simulink model "PrmM"  (R2025b)
settings: Solver=FixedStepDiscrete  StartTime=0.0  StopTime=5  RelTol=1e-3  EnableMultiTasking=on
PreLoadFcn:
  | loaded_model = bdroot;
  | cd (fileparts(get_param(bdroot,'FileName')));
  | SEGInitDevEnv
libraries: ParameterManager x2
settings Model: DataDictionary=PrmM_Data.sldd  EnableAccessToBaseWorkspace=off  Creator=BET2ST  LastModifiedBy=JVE2ST
settings DataIOCC: SaveFormat=StructureWithTime  SaveState=on
settings OptimizationCC: BlockReduction=off  DefaultParameterBehavior=Inlined  UseDivisionForNetSlopeComputation=on  DefaultUnderspecifiedDataType=single  InlineInvariantSignals=on  EnhancedBackFolding=on  PassReuseOutputArgsAs=Individual arguments  RollThreshold=40.0  ActiveStateOutputEnumStorageType=uint8  ZeroExternalMemoryAtStartup=off  EfficientFloat2IntCast=on  LifeSpan=inf  BufferReusableBoundary=off  OptimizeBlockOrder=speed  DifferentSizesBufferReuse=on  OptimizationCustomize=off  LabelGuidedReuse=on  EfficientTunableParamExpr=on
settings DebuggingCC: SignalInfNanChecking=error  SignalRangeChecking=error  ReadBeforeWriteMsg=EnableAllAsError  WriteAfterWriteMsg=EnableAllAsError  WriteAfterReadMsg=EnableAllAsError  AlgebraicLoopMsg=error  ArtificialAlgebraicLoopMsg=error  SaveWithDisabledLinksMsg=error  SaveWithParameterizedLinksMsg=error  BlockPriorityViolationMsg=error  SolverPrmCheckMsg=error  InheritedTsInSrcMsg=error  SingleTaskRateTransMsg=error  TasksWithSamePriorityMsg=error  SigSpecEnsureSampleTimeMsg=error  CheckMatrixSingularityMsg=error  IntegerOverflowMsg=error  ParameterUnderflowMsg=error  ParameterPrecisionLossMsg=error  ParameterTunabilityLossMsg=error  UnderSpecifiedDataTypeMsg=error  UnnecessaryDatatypeConvMsg=warning  VectorMatrixConversionMsg=error  SignalLabelMismatchMsg=error  UnconnectedInputMsg=error  UnconnectedOutputMsg=error  UnconnectedLineMsg=error  SFcnCompatibilityMsg=error  FrameProcessingCompatibilityMsg=warning  UniqueDataStoreMsg=error  BusObjectLabelMismatch=error  RootOutportRequireBusObject=error  AssertControl=DisableAll  AllowSymbolicDim=off  ModelReferenceIOMismatchMessage=error  UnknownTsInhSupMsg=error  ModelReferenceDataLoggingMessage=error  StateNameClashWarn=warning  StrictBusMsg=ErrorOnBusTreatedAsVector  NonBusSignalsTreatedAsBus=error  SFInvalidInputDataAccessInChartInitDiag=error  SFTransitionOutsideNaturalParentDiag=error  SFUnreachableExecutionPathDiag=error  SFUndirectedBroadcastEventsDiag=error  SFTransitionActionBeforeConditionDiag=error  SFTemporalDelaySmallerThanSampleTimeDiag=error  SFSelfTransitionDiag=error  SFExecutionAtInitializationDiag=error  IntegerSaturationMsg=error
settings HardwareCC: ProdBitPerPointer=32.0  ProdBitPerSizeT=32.0  ProdBitPerPtrDiffT=32.0  ProdLargestAtomicInteger=Long  ProdWordSize=32.0  ProdHWDeviceType=Infineon->TriCore
settings ModelReferenceCC: EnableRefExpFcnMdlSchedulingChecks=on  EnableParallelModelReferenceBuilds=on  ModelReferenceNumInstancesAllowed=Single  PropagateSignalLabelsOutOfModel=off
settings SFSimCC: SFSimEcho=off  SimGenImportedTypeDefs=on  CompileTimeRecursionLimit=0.0  EnableRuntimeRecursion=off  MATLABDynamicMemAlloc=off
settings RTWCC: SystemTargetFile=autosar.tlc  GenCodeOnly=on  TemplateMakefile=ert_default_tmf  PostCodeGenCommand=SEGPostCodeGenCallback(modelName, buildInfo)  DataTypeReplacement=CDataTypesFixedWidth  Description=AUTOSAR
settings CodeAppCC: ForceParamTrailComments=on  CommentStyle=Single-line  IgnoreCustomStorageClasses=off  IgnoreTestpoints=on  OperatorAnnotations=on  SimulinkDataObjDesc=on  SFDataObjDesc=on  MATLABFcnDesc=on  MangleLength=4.0  SharedChecksumLength=4.0  CustomSymbolStrGlobalVar=$U$R$N$M  CustomSymbolStrType=$R_$N$M  CustomSymbolStrFcn=$U$R_$N$F$M  CustomSymbolStrFcnArg=$U$N$M_$I[l]  CustomSymbolStrBlkIO=$N$M  InsertBlockDesc=on  StateflowObjectComments=on  MATLABSourceComments=on  ReqsInCode=on
settings STFCustomTargetCC: SystemTargetFile=autosar.tlc  TargetLangStandard=C99 (ISO)  UtilityFuncGeneration=Shared location  MultiwordLength=256.0  ParMdlRefBuildCompliant=on  CompOptLevelCompliant=on  ConcurrentExecutionCompliant=off  IncludeMdlTerminateFcn=off  CombineOutputUpdateFcns=on  SuppressErrorStatus=on  ERTCustomFileBanners=on  SubcomponentCodeInterfacePackaging=Nonreusable function  SupportNonFinite=off  SupportComplex=off  SupportContinuousTime=off  SupportNonInlinedSFcns=off  RemoveResetFunc=on  ParenthesesLevel=Standards  CastingMode=Standards  MATLABClassNameForMDSCustomization=Simulink.SoftwareTarget.ERTCustomization  AutosarCompliant=on  GRTInterface=off  UseToolchainInfoCompliant=on  GenerateSharedConstants=off  LookupTableObjectStructAxisOrder=2,1,3,4,...  LUTObjectStructOrderEvenSpacing=Size,Table,Breakpoints  AutosarSchemaVersion=R23-11  AutosarMaxShortNameLength=128.0  AutosarCompilerAbstraction=off  AutosarMatrixIOAsArray=off  DisableAUTOSARRoutinesHostLibrary=off
settings ERTTargetCC: ERTCustomFileTemplate=example_file_process.tlc  ERTFilePackagingFormat=Compact  PreserveExpressionOrder=on  SuppressUnreachableDefaultCases=off  EnableSignedLeftShifts=off  EnableSignedRightShifts=off  BooleanTrueId=TRUE  BooleanFalseId=FALSE  MemSecPackage=arMemmap  MemSecDataInternal=VAR_UNSPECIFIED  MemSecFuncExecute=CODE  MemSecFuncSharedUtil=CODE  TargetLangStandard=C99 (ISO)  UtilityFuncGeneration=Shared location  ConcurrentExecutionCompliant=off  IncludeMdlTerminateFcn=off  SuppressErrorStatus=on  SubcomponentCodeInterfacePackaging=Nonreusable function  SupportNonFinite=off  SupportComplex=off  ParenthesesLevel=Standards  CastingMode=Standards  ModelStepFunctionPrototypeControlCompliant=off  CPPClassGenCompliant=off  AutosarCompliant=on  GenerateSharedConstants=off  LookupTableObjectStructAxisOrder=2,1,3,4,...  LUTObjectStructOrderEvenSpacing=Size,Table,Breakpoints

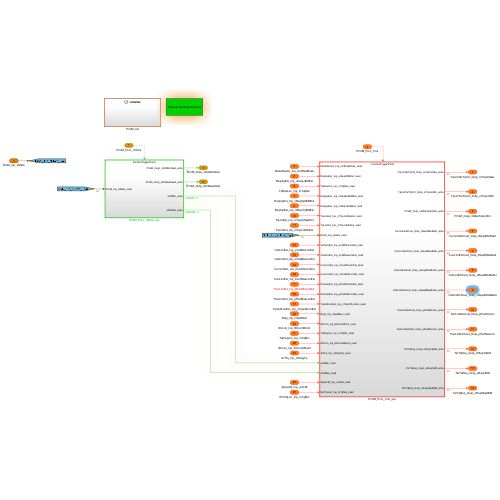
[thumbnail: Simulink's stored preview of the top-level diagram]
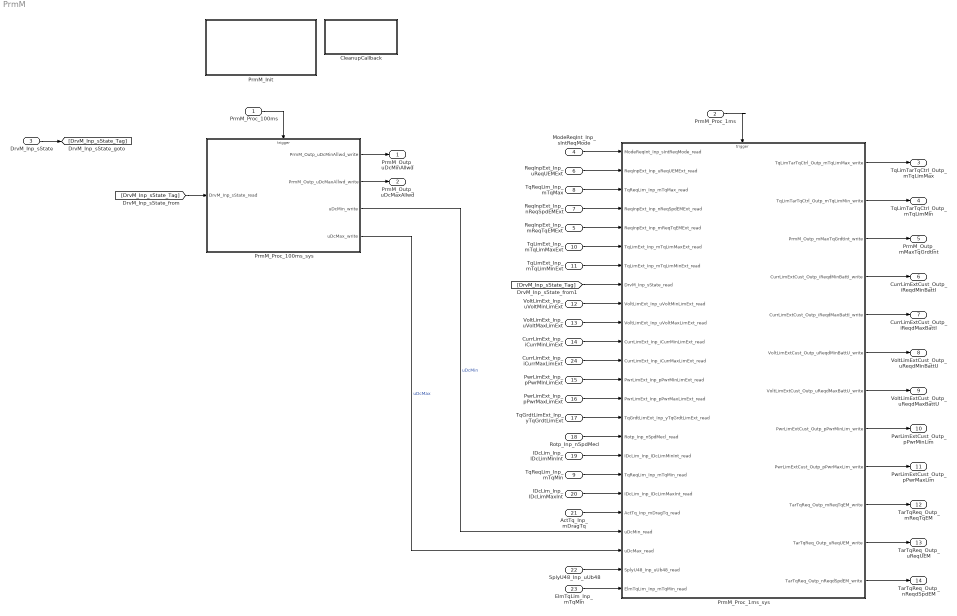
== system PrmM ==
  PrmM_Proc_100ms : Inport  SampleTime=0.1  OutputFunctionCall=on
  PrmM_Proc_1ms : Inport  Port=2  SampleTime=0.001  OutputFunctionCall=on
  DrvM_Inp_sState : Inport  Port=3  OutDataTypeStr=Enum: AD_DrvM_tSTATEIDX_E  PortDimensions=1
  ModeReqInt_Inp_sIntReqMode : Inport  Port=4  OutDataTypeStr=Enum: AD_DrvM_tSTATEIDX_E  PortDimensions=1
  ReqInpExt_Inp_mReqTqEMExt : Inport  Port=5  OutMin=-75  OutMax=75  OutDataTypeStr=AD_tMREQTQEMEXT  PortDimensions=1
  ReqInpExt_Inp_uReqUEMExt : Inport  Port=6  OutMin=0  OutMax=60  OutDataTypeStr=AD_tUREQVOLTEMEXT  PortDimensions=1
  ReqInpExt_Inp_nReqSpdEMExt : Inport  Port=7  OutMin=-10000  OutMax=55534  OutDataTypeStr=AD_tNREQDSPDEMEXT  PortDimensions=1
  TqReqLim_Inp_mTqMax : Inport  Port=8  OutMin=-85  OutMax=85  OutDataTypeStr=AD_TqReqLim_tMTQMAX  PortDimensions=1
  TqReqLim_Inp_mTqMin : Inport  Port=9  OutMin=-85  OutMax=85  OutDataTypeStr=AD_TqReqLim_tMTQMIN  PortDimensions=1
  TqLimExt_Inp_mTqLimMaxExt : Inport  Port=10  OutMin=0  OutMax=65  OutDataTypeStr=AD_tMTQLIMMAXEXT  PortDimensions=1
  TqLimExt_Inp_mTqLimMinExt : Inport  Port=11  OutMin=-65  OutMax=0  OutDataTypeStr=AD_tMTQLIMMINEXT  PortDimensions=1
  VoltLimExt_Inp_uVoltMinLimExt : Inport  Port=12  OutMin=20  OutMax=65  OutDataTypeStr=AD_tUVOLTMINLIMEXT  PortDimensions=1
  VoltLimExt_Inp_uVoltMaxLimExt : Inport  Port=13  OutMin=20  OutMax=65  OutDataTypeStr=AD_tUVOLTMAXLIMEXT  PortDimensions=1
  CurrLimExt_Inp_iCurrMinLimExt : Inport  Port=14  OutMin=-1200  OutMax=1200  OutDataTypeStr=AD_tICURRMINLIMEXT  PortDimensions=1
  PwrLimExt_Inp_pPwrMInLimExt : Inport  Port=15  OutMin=-16000  OutMax=16000  OutDataTypeStr=AD_tPPWRMINLIMEXT  PortDimensions=1
  PwrLimExt_Inp_pPwrMaxLimExt : Inport  Port=16  OutMin=-16000  OutMax=16000  OutDataTypeStr=AD_tPPWRMAXLIMEXT  PortDimensions=1
  TqGrdtLimExt_Inp_yTqGrdtLimExt : Inport  Port=17  OutMin=0  OutMax=2000  OutDataTypeStr=AD_tYTQGRDTLIMEXT  PortDimensions=1
  Rotp_Inp_nSpdMecl : Inport  Port=18  OutMin=-22000  OutMax=22000  OutDataTypeStr=AD_RotP_tNSPDMECL  PortDimensions=1
  IDcLim_Inp_IDcLimMinInt : Inport  Port=19  OutMin=-400  OutMax=0  OutDataTypeStr=AD_tIDCLIMMININT  PortDimensions=1
  IDcLim_Inp_IDcLimMaxInt : Inport  Port=20  OutMin=0  OutMax=400  OutDataTypeStr=AD_tIDCLIMMAXINT  PortDimensions=1
  ActTq_Inp_mDragTq : Inport  Port=21  OutMin=-85  OutMax=85  OutDataTypeStr=AD_ActTq_tMDRAGTQ  PortDimensions=1
  SplyU48_Inp_uUb48 : Inport  Port=22  OutMin=0  OutMax=80  OutDataTypeStr=AD_SplyU_tUUB48  PortDimensions=1
  ElmTqLim_Inp_mTqMin : Inport  Port=23  OutMin=-85  OutMax=0  OutDataTypeStr=AD_ElmTqLim_tMTQMIN  PortDimensions=1
  CurrLimExt_Inp_iCurrMaxLimExt : Inport  Port=24  OutMin=-1200  OutMax=1200  OutDataTypeStr=AD_tICURRMAXLIMEXT  PortDimensions=1
  CleanupCallback : Subsystem
      settings: OpenFcn=SEGCleanWorkspace
      mask Display: disp('Cleanup Working Directory')
  PrmM_Init : Subsystem
  PrmM_Proc_100ms_sys : Subsystem
  PrmM_Proc_1ms_sys : Subsystem
  PrmM_Outp_uDcMinAllwd : Outport  OutMin=20  OutMax=65  OutDataTypeStr=AD_PrmM_tUDCMINALLWD  PortDimensions=1  VectorParamsAs1DForOutWhenUnconnected=off
  PrmM_Outp_uDcMaxAllwd : Outport  Port=2  OutMin=20  OutMax=65  OutDataTypeStr=AD_PrmM_tUDCMAXALLWD  PortDimensions=1  VectorParamsAs1DForOutWhenUnconnected=off
  TqLimTarTqCtrl_Outp_mTqLimMax : Outport  Port=3  OutMin=-75  OutMax=75  OutDataTypeStr=AD_ComWrp_tMTQLIMMAX  PortDimensions=1  VectorParamsAs1DForOutWhenUnconnected=off
  TqLimTarTqCtrl_Outp_mTqLimMin : Outport  Port=4  OutMin=-75  OutMax=75  OutDataTypeStr=AD_ComWrp_tMTQLIMMIN  PortDimensions=1  VectorParamsAs1DForOutWhenUnconnected=off
  PrmM_Outp_mMaxTqGrdtInt : Outport  Port=5  OutMin=0.10000000149011612  OutMax=2000  OutDataTypeStr=AD_PrmM_tMMAXTQGRDINT  PortDimensions=1  VectorParamsAs1DForOutWhenUnconnected=off
  CurrLimExtCust_Outp_iReqdMinBattI : Outport  Port=6  OutMin=-1200  OutMax=1200  OutDataTypeStr=AD_ComWrp_tIREQDMINBATTI  PortDimensions=1  VectorParamsAs1DForOutWhenUnconnected=off
  CurrLimExtCust_Outp_iReqdMaxBattI : Outport  Port=7  OutMin=-1200  OutMax=1200  OutDataTypeStr=AD_ComWrp_tIREQDMAXBATTI  PortDimensions=1  VectorParamsAs1DForOutWhenUnconnected=off
  VoltLimExtCust_Outp_uReqdMinBattU : Outport  Port=8  OutMin=0  OutMax=2500  OutDataTypeStr=AD_ComWrp_tUREQDMINBATTU  PortDimensions=1  VectorParamsAs1DForOutWhenUnconnected=off
  VoltLimExtCust_Outp_uReqdMaxBattU : Outport  Port=9  OutMin=0  OutMax=2500  OutDataTypeStr=AD_ComWrp_tUREQDMAXBATTU  PortDimensions=1  VectorParamsAs1DForOutWhenUnconnected=off
  PwrLimExtCust_Outp_pPwrMinLim : Outport  Port=10  OutMin=-819000  OutMax=819200  OutDataTypeStr=AD_ComWrp_tPPWRMINLIM  PortDimensions=1  VectorParamsAs1DForOutWhenUnconnected=off
  PwrLimExtCust_Outp_pPwrMaxLim : Outport  Port=11  OutMin=-819000  OutMax=819200  OutDataTypeStr=AD_ComWrp_tPPWRMAXLIM  PortDimensions=1  VectorParamsAs1DForOutWhenUnconnected=off
  TarTqReq_Outp_mReqTqEM : Outport  Port=12  OutMin=-75  OutMax=75  OutDataTypeStr=AD_ComWrp_tMREQTQEM  PortDimensions=1  VectorParamsAs1DForOutWhenUnconnected=off
  TarTqReq_Outp_uReqUEM : Outport  Port=13  OutMin=0  OutMax=60  OutDataTypeStr=AD_ComWrp_tUREQVOLTEM  PortDimensions=1  VectorParamsAs1DForOutWhenUnconnected=off
  TarTqReq_Outp_nReqdSpdEM : Outport  Port=14  OutMin=-10000  OutMax=55534  OutDataTypeStr=AD_ComWrp_tNREQDSPDEM  PortDimensions=1  VectorParamsAs1DForOutWhenUnconnected=off
  wires:
  PrmM_Proc_100ms_sys/1(PrmM_Outp_uDcMinAllwd_write) -> PrmM_Outp_uDcMinAllwd/1
  PrmM_Proc_100ms_sys/2(PrmM_Outp_uDcMaxAllwd_write) -> PrmM_Outp_uDcMaxAllwd/1
  ModeReqInt_Inp_sIntReqMode/1 -> PrmM_Proc_1ms_sys/1(ModeReqInt_Inp_sIntReqMode_read)
  ReqInpExt_Inp_uReqUEMExt/1 -> PrmM_Proc_1ms_sys/2(ReqInpExt_Inp_uReqUEMExt_read)
  TqReqLim_Inp_mTqMax/1 -> PrmM_Proc_1ms_sys/3(TqReqLim_Inp_mTqMax_read)
  ReqInpExt_Inp_nReqSpdEMExt/1 -> PrmM_Proc_1ms_sys/4(ReqInpExt_Inp_nReqSpdEMExt_read)
  ReqInpExt_Inp_mReqTqEMExt/1 -> PrmM_Proc_1ms_sys/5(ReqInpExt_Inp_mReqTqEMExt_read)
  TqLimExt_Inp_mTqLimMaxExt/1 -> PrmM_Proc_1ms_sys/6(TqLimExt_Inp_mTqLimMaxExt_read)
  TqLimExt_Inp_mTqLimMinExt/1 -> PrmM_Proc_1ms_sys/7(TqLimExt_Inp_mTqLimMinExt_read)
  VoltLimExt_Inp_uVoltMinLimExt/1 -> PrmM_Proc_1ms_sys/9(VoltLimExt_Inp_uVoltMinLimExt_read)
  VoltLimExt_Inp_uVoltMaxLimExt/1 -> PrmM_Proc_1ms_sys/10(VoltLimExt_Inp_uVoltMaxLimExt_read)
  CurrLimExt_Inp_iCurrMinLimExt/1 -> PrmM_Proc_1ms_sys/11(CurrLimExt_Inp_iCurrMinLimExt_read)
  PwrLimExt_Inp_pPwrMInLimExt/1 -> PrmM_Proc_1ms_sys/13(PwrLimExt_Inp_pPwrMInLimExt_read)
  PwrLimExt_Inp_pPwrMaxLimExt/1 -> PrmM_Proc_1ms_sys/14(PwrLimExt_Inp_pPwrMaxLimExt_read)
  TqGrdtLimExt_Inp_yTqGrdtLimExt/1 -> PrmM_Proc_1ms_sys/15(TqGrdtLimExt_Inp_yTqGrdtLimExt_read)
  Rotp_Inp_nSpdMecl/1 -> PrmM_Proc_1ms_sys/16(Rotp_Inp_nSpdMecl_read)
  IDcLim_Inp_IDcLimMinInt/1 -> PrmM_Proc_1ms_sys/17(IDcLim_Inp_IDcLimMinInt_read)
  TqReqLim_Inp_mTqMin/1 -> PrmM_Proc_1ms_sys/18(TqReqLim_Inp_mTqMin_read)
  IDcLim_Inp_IDcLimMaxInt/1 -> PrmM_Proc_1ms_sys/19(IDcLim_Inp_IDcLimMaxInt_read)
  ActTq_Inp_mDragTq/1 -> PrmM_Proc_1ms_sys/20(ActTq_Inp_mDragTq_read)
  PrmM_Proc_1ms_sys/1(TqLimTarTqCtrl_Outp_mTqLimMax_write) -> TqLimTarTqCtrl_Outp_mTqLimMax/1
  PrmM_Proc_1ms_sys/2(TqLimTarTqCtrl_Outp_mTqLimMin_write) -> TqLimTarTqCtrl_Outp_mTqLimMin/1
  PrmM_Proc_1ms_sys/3(PrmM_Outp_mMaxTqGrdtInt_write) -> PrmM_Outp_mMaxTqGrdtInt/1
  PrmM_Proc_1ms_sys/4(CurrLimExtCust_Outp_iReqdMinBattI_write) -> CurrLimExtCust_Outp_iReqdMinBattI/1
  PrmM_Proc_1ms_sys/5(CurrLimExtCust_Outp_iReqdMaxBattI_write) -> CurrLimExtCust_Outp_iReqdMaxBattI/1
  PrmM_Proc_1ms_sys/6(VoltLimExtCust_Outp_uReqdMinBattU_write) -> VoltLimExtCust_Outp_uReqdMinBattU/1
  PrmM_Proc_1ms_sys/7(VoltLimExtCust_Outp_uReqdMaxBattU_write) -> VoltLimExtCust_Outp_uReqdMaxBattU/1
  PrmM_Proc_1ms_sys/8(PwrLimExtCust_Outp_pPwrMinLim_write) -> PwrLimExtCust_Outp_pPwrMinLim/1
  PrmM_Proc_1ms_sys/9(PwrLimExtCust_Outp_pPwrMaxLim_write) -> PwrLimExtCust_Outp_pPwrMaxLim/1
  PrmM_Proc_1ms_sys/10(TarTqReq_Outp_mReqTqEM_write) -> TarTqReq_Outp_mReqTqEM/1
  PrmM_Proc_1ms_sys/11(TarTqReq_Outp_uReqUEM_write) -> TarTqReq_Outp_uReqUEM/1
  PrmM_Proc_1ms_sys/12(TarTqReq_Outp_nReqdSpdEM_write) -> TarTqReq_Outp_nReqdSpdEM/1
  PrmM_Proc_100ms_sys/3(uDcMin_write) -> PrmM_Proc_1ms_sys/21(uDcMin_read)  "uDcMin"
  PrmM_Proc_100ms_sys/4(uDcMax_write) -> PrmM_Proc_1ms_sys/22(uDcMax_read)  "uDcMax"
  DrvM_Inp_sState/1 -> [DrvM_Inp_sState_Tag]
  [DrvM_Inp_sState_Tag] -> PrmM_Proc_100ms_sys/1(DrvM_Inp_sState_read)
  [DrvM_Inp_sState_Tag] -> PrmM_Proc_1ms_sys/8(DrvM_Inp_sState_read)
  PrmM_Proc_100ms/1 -> PrmM_Proc_100ms_sys/Trigger
  PrmM_Proc_1ms/1 -> PrmM_Proc_1ms_sys/Trigger
  SplyU48_Inp_uUb48/1 -> PrmM_Proc_1ms_sys/23(SplyU48_Inp_uUb48_read)
  ElmTqLim_Inp_mTqMin/1 -> PrmM_Proc_1ms_sys/24(ElmTqLim_Inp_mTqMin_read)
  CurrLimExt_Inp_iCurrMaxLimExt/1 -> PrmM_Proc_1ms_sys/12(CurrLimExt_Inp_iCurrMaxLimExt_read)

== system PrmM/CleanupCallback ==

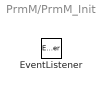
== system PrmM/PrmM_Init ==
  EventListener : EventListener  EventName=reset

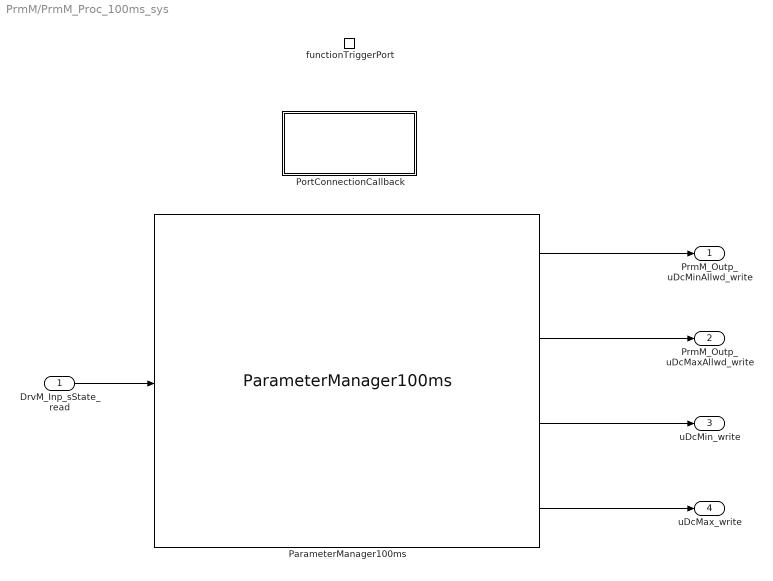
== system PrmM/PrmM_Proc_100ms_sys ==
  DrvM_Inp_sState_read : Inport
  functionTriggerPort : TriggerPort  TriggerType=function-call  VariantControl=(inherit)  SampleTimeType=periodic  SampleTime=-1
      settings: AttributesFormatString=|
      | SampleTime=%<SampleTime>
      | SampleTimeType=%<SampleTimeType>
      | StatesWhenEnabling=%<StatesWhenEnabling>
  ParameterManager100ms : ParameterManager/ParameterManager100ms  SystemSampleTime=-1  VariantActivationTime=update diagram  EmptyChoice=off  PassThrough=off  PassThroughVariantControl=(default)  EmptyChoiceVariantControl=(default)  AllowFlexibleInterface=on  Latency=0  AutoFrameSizeCalculation=off
  PortConnectionCallback : Subsystem
      settings: OpenFcn=SEGPortConnectionCallback
      mask Display: disp('Connect detected Ports')
  PrmM_Outp_uDcMinAllwd_write : Outport  VectorParamsAs1DForOutWhenUnconnected=off
      settings: EnsureOutportIsVirtual=on
  PrmM_Outp_uDcMaxAllwd_write : Outport  Port=2  VectorParamsAs1DForOutWhenUnconnected=off
      settings: EnsureOutportIsVirtual=on
  uDcMin_write : Outport  Port=3  OutMin=20  OutMax=65  OutDataTypeStr=AD_PrmM_tUDCMINALLWD  PortDimensions=1  VectorParamsAs1DForOutWhenUnconnected=off
  uDcMax_write : Outport  Port=4  OutMin=20  OutMax=65  OutDataTypeStr=AD_PrmM_tUDCMAXALLWD  PortDimensions=1  VectorParamsAs1DForOutWhenUnconnected=off
  wires:
  ParameterManager100ms/1 -> PrmM_Outp_uDcMinAllwd_write/1
  ParameterManager100ms/2 -> PrmM_Outp_uDcMaxAllwd_write/1
  ParameterManager100ms/3 -> uDcMin_write/1
  ParameterManager100ms/4 -> uDcMax_write/1
  DrvM_Inp_sState_read/1 -> ParameterManager100ms/1

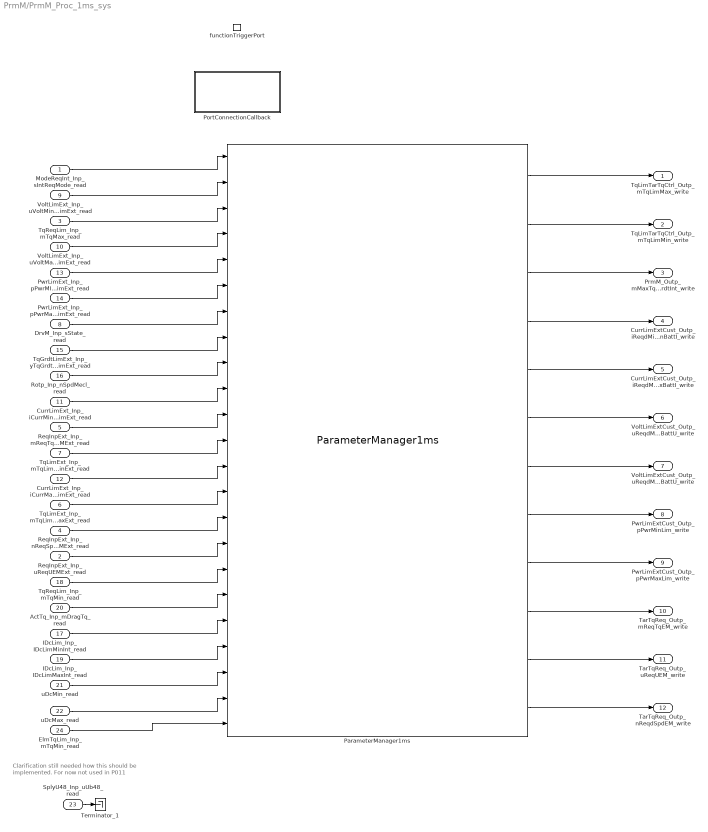
== system PrmM/PrmM_Proc_1ms_sys ==
  note: Clarification still needed how
      | this should be implemented.
      | For now not used in P011
  ModeReqInt_Inp_sIntReqMode_read : Inport
  ReqInpExt_Inp_uReqUEMExt_read : Inport  Port=2
  TqReqLim_Inp_mTqMax_read : Inport  Port=3
  ReqInpExt_Inp_nReqSpdEMExt_read : Inport  Port=4
  ReqInpExt_Inp_mReqTqEMExt_read : Inport  Port=5
  TqLimExt_Inp_mTqLimMaxExt_read : Inport  Port=6
  TqLimExt_Inp_mTqLimMinExt_read : Inport  Port=7
  DrvM_Inp_sState_read : Inport  Port=8
  VoltLimExt_Inp_uVoltMinLimExt_read : Inport  Port=9
  VoltLimExt_Inp_uVoltMaxLimExt_read : Inport  Port=10
  CurrLimExt_Inp_iCurrMinLimExt_read : Inport  Port=11
  CurrLimExt_Inp_iCurrMaxLimExt_read : Inport  Port=12
  PwrLimExt_Inp_pPwrMInLimExt_read : Inport  Port=13
  PwrLimExt_Inp_pPwrMaxLimExt_read : Inport  Port=14
  TqGrdtLimExt_Inp_yTqGrdtLimExt_read : Inport  Port=15
  Rotp_Inp_nSpdMecl_read : Inport  Port=16
  IDcLim_Inp_IDcLimMinInt_read : Inport  Port=17
  TqReqLim_Inp_mTqMin_read : Inport  Port=18
  IDcLim_Inp_IDcLimMaxInt_read : Inport  Port=19
  ActTq_Inp_mDragTq_read : Inport  Port=20
  uDcMin_read : Inport  Port=21
  uDcMax_read : Inport  Port=22
  SplyU48_Inp_uUb48_read : Inport  Port=23
  ElmTqLim_Inp_mTqMin_read : Inport  Port=24
  functionTriggerPort : TriggerPort  TriggerType=function-call  VariantControl=(inherit)  SampleTimeType=periodic  SampleTime=-1
      settings: AttributesFormatString=|
      | SampleTime=%<SampleTime>
      | SampleTimeType=%<SampleTimeType>
      | StatesWhenEnabling=%<StatesWhenEnabling>
  ParameterManager1ms : ParameterManager/ParameterManager1ms  SystemSampleTime=-1  VariantActivationTime=update diagram  EmptyChoice=off  PassThrough=off  PassThroughVariantControl=(default)  EmptyChoiceVariantControl=(default)  AllowFlexibleInterface=on  Latency=0  AutoFrameSizeCalculation=off
  PortConnectionCallback : Subsystem
      settings: OpenFcn=SEGPortConnectionCallback
      mask Display: disp('Connect detected Ports')
  Terminator_1 : Terminator
  TqLimTarTqCtrl_Outp_mTqLimMax_write : Outport  VectorParamsAs1DForOutWhenUnconnected=off
      settings: EnsureOutportIsVirtual=on
  TqLimTarTqCtrl_Outp_mTqLimMin_write : Outport  Port=2  VectorParamsAs1DForOutWhenUnconnected=off
      settings: EnsureOutportIsVirtual=on
  PrmM_Outp_mMaxTqGrdtInt_write : Outport  Port=3  VectorParamsAs1DForOutWhenUnconnected=off
      settings: EnsureOutportIsVirtual=on
  CurrLimExtCust_Outp_iReqdMinBattI_write : Outport  Port=4  VectorParamsAs1DForOutWhenUnconnected=off
      settings: EnsureOutportIsVirtual=on
  CurrLimExtCust_Outp_iReqdMaxBattI_write : Outport  Port=5  VectorParamsAs1DForOutWhenUnconnected=off
      settings: EnsureOutportIsVirtual=on
  VoltLimExtCust_Outp_uReqdMinBattU_write : Outport  Port=6  VectorParamsAs1DForOutWhenUnconnected=off
      settings: EnsureOutportIsVirtual=on
  VoltLimExtCust_Outp_uReqdMaxBattU_write : Outport  Port=7  VectorParamsAs1DForOutWhenUnconnected=off
      settings: EnsureOutportIsVirtual=on
  PwrLimExtCust_Outp_pPwrMinLim_write : Outport  Port=8  VectorParamsAs1DForOutWhenUnconnected=off
      settings: EnsureOutportIsVirtual=on
  PwrLimExtCust_Outp_pPwrMaxLim_write : Outport  Port=9  VectorParamsAs1DForOutWhenUnconnected=off
      settings: EnsureOutportIsVirtual=on
  TarTqReq_Outp_mReqTqEM_write : Outport  Port=10  VectorParamsAs1DForOutWhenUnconnected=off
      settings: EnsureOutportIsVirtual=on
  TarTqReq_Outp_uReqUEM_write : Outport  Port=11  VectorParamsAs1DForOutWhenUnconnected=off
      settings: EnsureOutportIsVirtual=on
  TarTqReq_Outp_nReqdSpdEM_write : Outport  Port=12  VectorParamsAs1DForOutWhenUnconnected=off
      settings: EnsureOutportIsVirtual=on
  wires:
  ModeReqInt_Inp_sIntReqMode_read/1 -> ParameterManager1ms/1
  TqReqLim_Inp_mTqMax_read/1 -> ParameterManager1ms/3
  DrvM_Inp_sState_read/1 -> ParameterManager1ms/7
  Rotp_Inp_nSpdMecl_read/1 -> ParameterManager1ms/9
  TqReqLim_Inp_mTqMin_read/1 -> ParameterManager1ms/17
  ActTq_Inp_mDragTq_read/1 -> ParameterManager1ms/18
  ParameterManager1ms/1 -> TqLimTarTqCtrl_Outp_mTqLimMax_write/1
  ParameterManager1ms/2 -> TqLimTarTqCtrl_Outp_mTqLimMin_write/1
  ParameterManager1ms/3 -> PrmM_Outp_mMaxTqGrdtInt_write/1
  ParameterManager1ms/4 -> CurrLimExtCust_Outp_iReqdMinBattI_write/1
  ParameterManager1ms/5 -> CurrLimExtCust_Outp_iReqdMaxBattI_write/1
  ParameterManager1ms/6 -> VoltLimExtCust_Outp_uReqdMinBattU_write/1
  ParameterManager1ms/7 -> VoltLimExtCust_Outp_uReqdMaxBattU_write/1
  ParameterManager1ms/8 -> PwrLimExtCust_Outp_pPwrMinLim_write/1
  ParameterManager1ms/9 -> PwrLimExtCust_Outp_pPwrMaxLim_write/1
  ParameterManager1ms/10 -> TarTqReq_Outp_mReqTqEM_write/1
  ParameterManager1ms/11 -> TarTqReq_Outp_uReqUEM_write/1
  ParameterManager1ms/12 -> TarTqReq_Outp_nReqdSpdEM_write/1
  uDcMax_read/1 -> ParameterManager1ms/22
  uDcMin_read/1 -> ParameterManager1ms/21
  IDcLim_Inp_IDcLimMaxInt_read/1 -> ParameterManager1ms/20
  IDcLim_Inp_IDcLimMinInt_read/1 -> ParameterManager1ms/19
  VoltLimExt_Inp_uVoltMinLimExt_read/1 -> ParameterManager1ms/2
  VoltLimExt_Inp_uVoltMaxLimExt_read/1 -> ParameterManager1ms/4
  PwrLimExt_Inp_pPwrMInLimExt_read/1 -> ParameterManager1ms/5
  CurrLimExt_Inp_iCurrMinLimExt_read/1 -> ParameterManager1ms/10
  CurrLimExt_Inp_iCurrMaxLimExt_read/1 -> ParameterManager1ms/13
  PwrLimExt_Inp_pPwrMaxLimExt_read/1 -> ParameterManager1ms/6
  TqLimExt_Inp_mTqLimMinExt_read/1 -> ParameterManager1ms/12
  TqLimExt_Inp_mTqLimMaxExt_read/1 -> ParameterManager1ms/14
  ReqInpExt_Inp_mReqTqEMExt_read/1 -> ParameterManager1ms/11
  ReqInpExt_Inp_uReqUEMExt_read/1 -> ParameterManager1ms/16
  ReqInpExt_Inp_nReqSpdEMExt_read/1 -> ParameterManager1ms/15
  TqGrdtLimExt_Inp_yTqGrdtLimExt_read/1 -> ParameterManager1ms/8
  SplyU48_Inp_uUb48_read/1 -> Terminator_1/1
  ElmTqLim_Inp_mTqMin_read/1 -> ParameterManager1ms/23

== system PrmM/PrmM_Proc_100ms_sys/PortConnectionCallback ==

== system PrmM/PrmM_Proc_1ms_sys/PortConnectionCallback ==
